simulink model "gantry_truth"  (R2025a)
settings: Solver=ode4  StartTime=0.0  StopTime=t(end)  FixedStep=ts  RelTol=1e-4  AbsTol=1e-8
undefined symbols (not defined in the file): ca, cb1, cb2, cc1, cc2, ccy, cg1, cg2, cy, d, g_fric, Jb, Jh, ka, kb1, kb2, L0, Lb, m1, m2, ma, mb, mh, P, ts, Y
libraries: cstblocks x1
settings Model: Creator=cocuser  LastModifiedBy=20203253
settings DataIOCC: ReturnWorkspaceOutputs=off

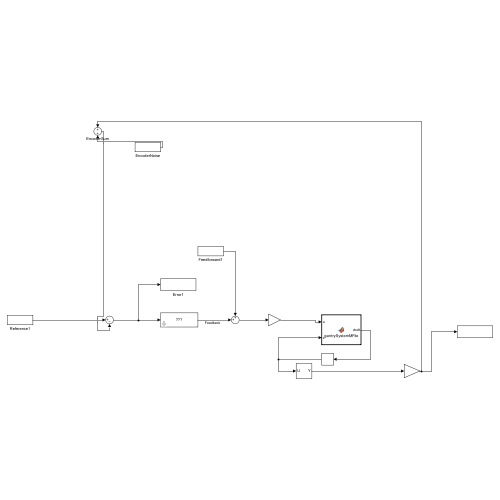
[thumbnail: Simulink's stored preview of the top-level diagram]
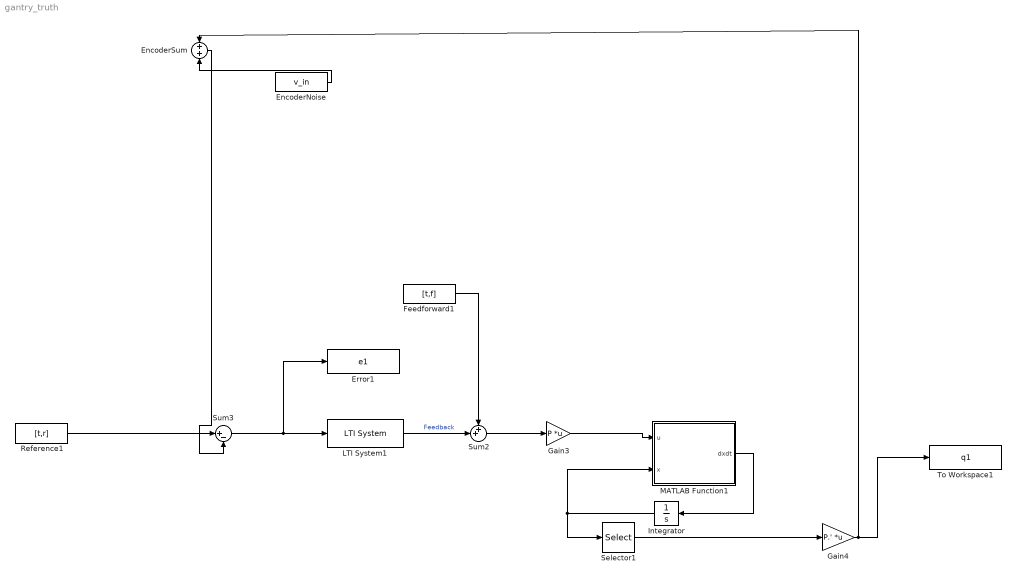
== system gantry_truth ==
  EncoderNoise : FromWorkspace  VariableName=v_in  SampleTime=ts  Interpolate=off  OutputAfterFinalValue=Holding final value
  EncoderSum : Sum
  Error1 : ToWorkspace  VariableName=e1  SampleTime=ts
  Feedforward1 : FromWorkspace  VariableName=[t,f]  SampleTime=ts
  Gain3 : Gain  Gain=P  Multiplication=Matrix(K*u)
  Gain4 : Gain  Gain=P.'  Multiplication=Matrix(K*u)
  Integrator : Integrator  InitialCondition=[0; 0; Y; 0; 0; 0; 0; 0]
  LTI System1 : cstblocks/LTI System  sys=Cfb  IC=[]  PadeOrder=0
  MATLAB Function1 : MATLAB Function  TreatAsAtomicUnit=on
  Reference1 : FromWorkspace  VariableName=[t,r]  SampleTime=ts
  Selector1 : Selector  InputPortWidth=8  IndexOptions=Index vector (dialog)  Indices=[1 2 3]  OutputSizes=1
  Sum2 : Sum  Inputs=++|
  Sum3 : Sum  Inputs=|+-
  To Workspace1 : ToWorkspace  VariableName=q1  SampleTime=ts
  wires:
  LTI System1/1 -> Sum2/2  "Feedback"
  Feedforward1/1 -> Sum2/1
  Sum3/1 -> Error1/1, LTI System1/1
  Integrator/1 -> MATLAB Function1/2(x), Selector1/1
  Selector1/1 -> Gain4/1
  Sum2/1 -> Gain3/1
  Gain3/1 -> MATLAB Function1/1(u)
  Gain4/1 -> To Workspace1/1, EncoderSum/1
  MATLAB Function1/1(dxdt) -> Integrator/1
  Reference1/1 -> Sum3/1
  EncoderNoise/1 -> EncoderSum/2
  EncoderSum/1 -> Sum3/2

== matlab function gantry_truth/MATLAB Function1 ==
  data: dxdt output; u input; x input; m1 parameter; m2 parameter; mb parameter; mh parameter; Jb parameter; Jh parameter; d parameter; Lb parameter; kb1 parameter; kb2 parameter; cg1 parameter; cg2 parameter; cb1 parameter; cb2 parameter; cy parameter; ma parameter; ka parameter; ca parameter; L0 parameter; cc1 parameter; cc2 parameter; ccy parameter; g_fric parameter
function dxdt = gantrySystemMFile(u,x,m1,m2,mb,mh,Jb,Jh,d,Lb,kb1,kb2,cg1,cg2,cb1,cb2,cy,ma,ka,ca,L0,cc1,cc2,ccy,g_fric)
dxdt = zeros(8,1);
dxdt = gantrySystemExtendedTanh(u,x,m1,m2,mb,mh,Lb,Jb,Jh,d,cg1,cg2,cb1,cb2,cy,kb1,kb2,ma,ka,ca,L0,cc1,cc2,ccy,g_fric);
end
